simulink model "QDrone_Capture"  (R2019a)
settings: Solver=ode2  StartTime=0.0  StopTime=inf  FixedStep=0.001  RelTol=1e-3  EnableMultiTasking=on
InitFcn:
  | p=fileparts(get_param('QDrone_Capture','FileName'));addpath(fullfile(p,'capture_tool'),fullfile(p,'optical_flow'));
values from neighbouring files (symbols this model uses):
  x = xp + K*(z-xp(1))    [qdrone_baro_height_kalman.m]    (also in qdrone_baro_height_kalman_smooth.m)
libraries: quarc_library x5
settings Model: SimulationMode=external  ExtModeTrigDuration=10000  Creator=user  LastModifiedBy=user
settings SolverCC: PositivePriorityOrder=on
settings DataIOCC: LimitDataPoints=on  SaveFormat=Array  ReturnWorkspaceOutputs=off
settings OptimizationCC: LifeSpan=inf
settings DebuggingCC: SolverPrmCheckMsg=warning  SFUnexpectedBacktrackingDiag=warning  SFNoUnconditionalDefaultTransitionDiag=warning  SFExecutionAtInitializationDiag=none  ArithmeticOperatorsInVariantConditions=warning
settings HardwareCC: ProdBitPerLong=64  ProdLargestAtomicFloat=None  ProdHWDeviceType=Intel->x86-64
settings ModelReferenceCC: PropagateSignalLabelsOutOfModel=off
settings SFSimCC: SimUseLocalCustomCode=off
settings RTWCC: SystemTargetFile=quarc_linux_x64.tlc  TemplateMakefile=quarc_linux_x64_tmf  Description=QUARC Linux x64 Target  RTWUseLocalCustomCode=off
settings CodeAppCC: StateflowObjectComments=on
settings STFCustomTargetCC: TargetLibSuffix=.a  TargetPreCompLibLocation=C:\PROGRA~3\QUARC\lib\2019a\LINUX_~1\release  ConcurrentExecutionCompliant=on  SystemTargetFile=quarc_linux_x64.tlc
settings GRTTargetCC: TargetLibSuffix=.a  TargetPreCompLibLocation=C:\PROGRA~3\QUARC\lib\2019a\LINUX_~1\release  TargetLangStandard=C89/C90 (ANSI)  ParMdlRefBuildCompliant=off  CompOptLevelCompliant=off  CombineOutputUpdateFcns=off  MatFileLogging=off  CPPClassGenCompliant=off  GRTInterface=on  UseToolchainInfoCompliant=off  ExtMode=on  ExtModeMexFile=quarc_comm  ExtModeMexArgs='-w -d /tmp -uri %u','tcpip://192.168.2.52:17005'
settings ConfigComp: CovMetricSettings=dw  CovHtmlReporting=on  CovSaveCumulativeToWorkspaceVar=on  CovSaveSingleToWorkspaceVar=on  CovExternalEMLEnable=off  CovSFcnEnable=off

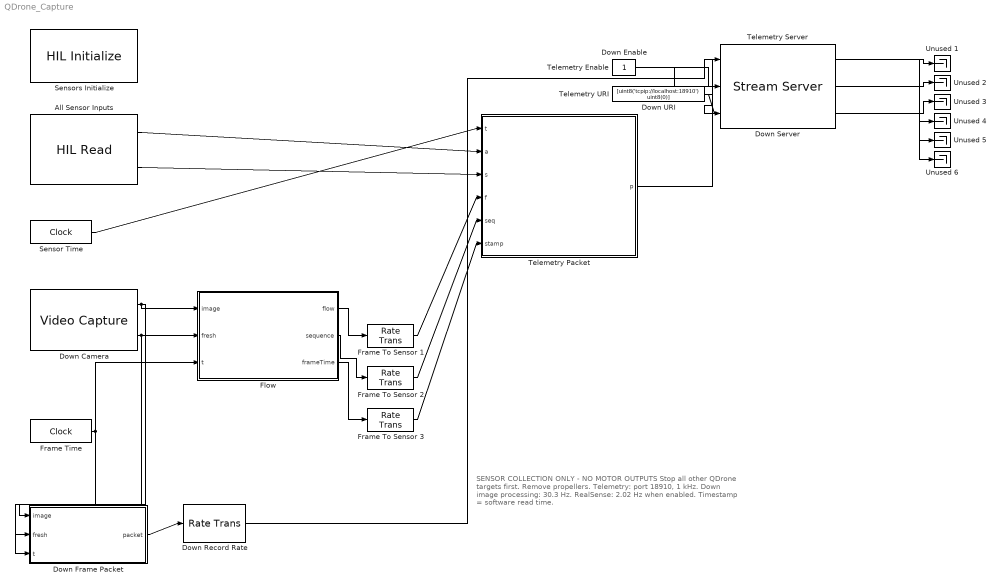
== system QDrone_Capture ==
  note: SENSOR COLLECTION ONLY - NO MOTOR OUTPUTS
      | Stop all other QDrone targets first. Remove propellers.
      | Telemetry: port 18910, 1 kHz. Down image processing: 30.3 Hz.
      | RealSense: 2.02 Hz when enabled. Timestamp = software read time.
  All Sensor Inputs : quarc_library/Data Acquisition/Generic/Immediate I//O/HIL Read  Priority=1  object_name=CaptureSensors  analog_channels=0:4  encoder_channels=[]  digital_channels=[]  other_channels=[3000:3002 4000:4002]  sample_time=0.001  active=on  vector_output=on  data_type_mode=Inherit via back propagation  encoder_data_type=double  digital_data_type=boolean
      settings: SourceProductName=The database C:\Users\user\AppData\Roaming\MathWorks\MATLAB\R2017a\slblocks_master.db is locked, or a table in the database is locked. (database is locked)
  Down Camera : quarc_library/Multimedia/Video Capture  source=device  device=2  filename=sample_movie.mov  value=[0 0; 0 0]  resolution=640 x 480  width=640  height=480  output_format=MATLAB greyscale (HxW)  data_type=uint8  sample_time=0.033  brightness_override=off  brightness=50.0  contrast_override=off  contrast=50.0  hue_override=off  hue=50.0  saturation_override=off  saturation=50.0  sharpness_override=off  sharpness=50.0  gamma_override=off  gamma=50.0  coloreffect_override=off  coloreffect=None  whitebalance_override=off  whitebalance=50.0  backlightcompensation_override=off  backlightcompensation=0.0  gain_override=off  gain=50.0  pan_override=off  pan=50.0  tilt_override=off  tilt=50.0  roll_override=off  roll=50.0  zoom_override=off  zoom=0.0  exposure_override=off  exposure=50.0  iris_override=off  iris=50.0  focus_override=off  focus=0.0
      settings: SourceProductName=QUARC Targets
  Down Enable : Constant
  Down Frame Packet : MATLAB Function  TreatAsAtomicUnit=on
  Down Record Rate : RateTransition  OutPortSampleTime=0.099
  Down Server : quarc_library/Communications/Basic/Stream Server  uri_source=External input port  uri=tcpip://localhost:18911  apply_uri_to_all_configs=on  send_buffer_size=614520  receive_buffer_size=1024  byte_order=little endian (Intel - LSB first)  optimization=Minimum latency  send_options=Send all data  receive_options=Do not receive data  default_value=[0]  sample_time=0.099  active=on  implementation=Use blocking I/O in a separate thread  send_fifo_size=8  receive_fifo_size=1000  send_priority=0  receive_priority=0  send_dimensions=off  receive_dimensions=off  max_dimensions=-1  data_type=Inherited via back propagation  type_expr=BusObject
  Down URI : Constant  Value=[uint8('tcpip://localhost:18911') uint8(0)]
  Flow : MATLAB Function  TreatAsAtomicUnit=on
  Frame Time : DigitalClock  SampleTime=0.033
  Frame To Sensor 1 : RateTransition  OutPortSampleTime=0.001
  Frame To Sensor 2 : RateTransition  OutPortSampleTime=0.001
  Frame To Sensor 3 : RateTransition  OutPortSampleTime=0.001
  Sensor Time : DigitalClock  SampleTime=0.001
  Sensors Initialize : quarc_library/Data Acquisition/Generic/Configuration/HIL Initialize  object_name=CaptureSensors  board_type=qdrone  board_number=0  board_options=gyro_fs=2000;gyro_rate=1000;gyro_os=4;accel_fs=16;accel_rate=400;accel_os=4;baro_os=4096  exclusive=on  active=on  hardware_clocks=[]  clock_modes=[]  initial_clock_frequencies=[]  set_clock_params_at_start=off  set_clock_params_at_switch_in=off  set_clock_frequencies_at_start=off  set_clock_frequencies_at_switch_in=off  analog_input_channels=[0:4]  analog_input_configurations=[]  analog_input_maximums=[3.3]  analog_input_minimums=[0]  set_analog_input_params_at_start=off  set_analog_input_params_at_switch_in=off  analog_output_channels=[]  analog_output_maximums=[]  analog_output_minimums=[]  initial_analog_outputs=[]  final_analog_outputs=[]  watchdog_analog_outputs=[]  set_analog_output_params_at_start=off  set_analog_output_params_at_switch_in=off  set_analog_outputs_at_start=off  set_analog_outputs_at_switch_in=off  set_analog_outputs_at_terminate=off  set_analog_outputs_at_switch_out=off  set_analog_outputs_on_watchdog=off  digital_input_channels=[]  digital_output_channels=[]  digital_output_configuration=[]  initial_digital_outputs=[0]  final_digital_outputs=[0]  watchdog_digital_outputs=[]  set_digital_output_params_at_start=off  set_digital_output_params_at_switch_in=off  set_digital_outputs_at_start=off  set_digital_outputs_at_switch_in=off  set_digital_outputs_at_terminate=off  set_digital_outputs_at_switch_out=off  set_digital_outputs_on_watchdog=off  encoder_channels=[]  quadrature=[4]  encoder_filter_frequency=50e6/1  initial_encoder_counts=[0]  set_encoder_params_at_start=off  set_encoder_params_at_switch_in=off  set_encoder_counts_at_start=off  set_encoder_counts_at_switch_in=off  pwm_channels=[]  pwm_modes=[4]  pwm_frequency=2000  pwm_configuration=[0]  pwm_alignment=[0]  pwm_polarity=[1]  pwm_leading_deadband=[]  pwm_trailing_deadband=[]  initial_pwm_outputs=[0]  final_pwm_outputs=[0]  watchdog_pwm_outputs=[0]  set_pwm_params_at_start=off  set_pwm_params_at_switch_in=off  set_pwm_outputs_at_start=off  set_pwm_outputs_at_switch_in=off  set_pwm_outputs_at_terminate=off  set_pwm_outputs_at_switch_out=off  set_pwm_outputs_on_watchdog=off  other_output_channels=[]  initial_other_outputs=[]  final_other_outputs=[]  watchdog_other_outputs=[]  set_other_outputs_at_start=off  set_other_outputs_at_switch_in=off  set_other_outputs_at_terminate=off  set_other_outputs_at_switch_out=off  set_other_outputs_on_watchdog=off
      settings: SourceProductName=The database C:\Users\user\AppData\Roaming\MathWorks\MATLAB\R2017a\slblocks_master.db is locked, or a table in the database is locked. (database is locked)
  Telemetry Enable : Constant
  Telemetry Packet : MATLAB Function  TreatAsAtomicUnit=on
  Telemetry Server : quarc_library/Communications/Basic/Stream Server  uri_source=External input port  uri=tcpip://localhost:18910  apply_uri_to_all_configs=on  send_buffer_size=65536  receive_buffer_size=1024  byte_order=little endian (Intel - LSB first)  optimization=Minimum latency  send_options=Send all data  receive_options=Do not receive data  default_value=[0]  sample_time=0.001  active=on  implementation=Use blocking I/O in a separate thread  send_fifo_size=20000  receive_fifo_size=1000  send_priority=0  receive_priority=0  send_dimensions=off  receive_dimensions=off  max_dimensions=-1  data_type=Inherited via back propagation  type_expr=BusObject
  Telemetry URI : Constant  Value=[uint8('tcpip://localhost:18910') uint8(0)]
  Unused {1..6} (6 alike) : Terminator
  wires:
  Down Camera/1 -> Flow/1(image), Down Frame Packet/1(image)
  Down Camera/2 -> Flow/2(fresh), Down Frame Packet/2(fresh)
  Frame Time/1 -> Flow/3(t), Down Frame Packet/3(t)
  Flow/1(flow) -> Frame To Sensor 1/1
  Flow/2(sequence) -> Frame To Sensor 2/1
  Flow/3(frameTime) -> Frame To Sensor 3/1
  Sensor Time/1 -> Telemetry Packet/1(t)
  All Sensor Inputs/1 -> Telemetry Packet/2(a)
  All Sensor Inputs/2 -> Telemetry Packet/3(s)
  Frame To Sensor 1/1 -> Telemetry Packet/4(f)
  Frame To Sensor 2/1 -> Telemetry Packet/5(seq)
  Frame To Sensor 3/1 -> Telemetry Packet/6(stamp)
  Telemetry Packet/1(p) -> Telemetry Server/1
  Telemetry Enable/1 -> Telemetry Server/2
  Telemetry URI/1 -> Telemetry Server/3
  Down Frame Packet/1(packet) -> Down Record Rate/1
  Down Record Rate/1 -> Down Server/1
  Down Enable/1 -> Down Server/2
  Down URI/1 -> Down Server/3
  Down Server/1 -> Unused 1/1
  Down Server/2 -> Unused 2/1
  Down Server/3 -> Unused 3/1
  Telemetry Server/1 -> Unused 4/1
  Telemetry Server/2 -> Unused 5/1
  Telemetry Server/3 -> Unused 6/1

== matlab function QDrone_Capture/Telemetry Packet ==
  data: t input; p output; a input; s input; f input; seq input; stamp input
function p=run(t,a,s,f,seq,stamp)
%#codegen
p=qdrone_capture_packet(t,a,s,f,seq,stamp);
end

== matlab function QDrone_Capture/Flow ==
  data: image input; flow output; fresh input; t input; sequence output; frameTime output
function [flow,sequence,frameTime]=run(image,fresh,t)
%#codegen
[flow,sequence,frameTime]=qdrone_capture_flow(image,fresh,t);
end

== matlab function QDrone_Capture/Down Frame Packet ==
  data: image input uint8 size=[480 640]; packet output uint8 size=[307260 1]; fresh input boolean; t input
function packet=run(image,fresh,t)
%#codegen
packet=qdrone_capture_frame(image,fresh,t,1);
end
